simulink model "HVAC_Control_SWC_AUTOSAR_v3_FaultHandling"  (R2022b)
settings: Solver=FixedStepDiscrete  StartTime=0  StopTime=70  FixedStep=0.1  RelTol=1e-3
settings Model: Creator=Utilisateur  LastModifiedBy=Utilisateur
settings DataIOCC: ExternalInput=hvacInputs_SILV3_02  LoadExternalInput=on
settings OptimizationCC: DefaultParameterBehavior=Inlined  UseDivisionForNetSlopeComputation=on  GainParamInheritBuiltInType=on  UseFloatMulNetSlope=on  InlineInvariantSignals=on  EnhancedBackFolding=on  PassReuseOutputArgsAs=Individual arguments  ZeroExternalMemoryAtStartup=off  ZeroInternalMemoryAtStartup=off  NoFixptDivByZeroProtection=on  EfficientFloat2IntCast=on  OptimizeBlockOrder=speed  DifferentSizesBufferReuse=on  OptimizationCustomize=off  EfficientTunableParamExpr=on
settings DebuggingCC: ParameterTunabilityLossMsg=error
settings HardwareCC: ProdLongLongMode=on
settings SFSimCC: MATLABDynamicMemAlloc=off
settings RTWCC: Description=AUTOSAR  SystemTargetFile=autosar.tlc  GenCodeOnly=on  TemplateMakefile=ert_default_tmf
settings CodeAppCC: ForceParamTrailComments=on  IgnoreCustomStorageClasses=off  OperatorAnnotations=on  SimulinkDataObjDesc=on  SFDataObjDesc=on  CustomSymbolStrGlobalVar=rt$N$M  CustomSymbolStrType=$N$M  CustomSymbolStrFcn=$N$M$F  CustomSymbolStrMacro=$N$M  InsertBlockDesc=on
settings STFCustomTargetCC: TargetLangStandard=C99 (ISO)  MultiwordLength=256  ParMdlRefBuildCompliant=on  CompOptLevelCompliant=on  IncludeMdlTerminateFcn=off  CombineOutputUpdateFcns=on  SuppressErrorStatus=on  ERTCustomFileBanners=on  SupportComplex=off  SupportContinuousTime=off  SupportNonInlinedSFcns=off  RemoveResetFunc=on  MATLABClassNameForMDSCustomization=Simulink.SoftwareTarget.ERTCustomization  AutosarCompliant=on  UseToolchainInfoCompliant=on  LookupTableObjectStructAxisOrder=2,1,3,4,...  LUTObjectStructOrderEvenSpacing=Size,Table,Breakpoints  SystemTargetFile=autosar.tlc
settings ERTTargetCC: TargetLangStandard=C99 (ISO)  ConcurrentExecutionCompliant=off  IncludeMdlTerminateFcn=off  SuppressErrorStatus=on  SupportComplex=off  ModelStepFunctionPrototypeControlCompliant=off  CPPClassGenCompliant=off  AutosarCompliant=on  LookupTableObjectStructAxisOrder=2,1,3,4,...  LUTObjectStructOrderEvenSpacing=Size,Table,Breakpoints  InlinedParameterPlacement=NonHierarchical  ERTCustomFileTemplate=example_file_process.tlc

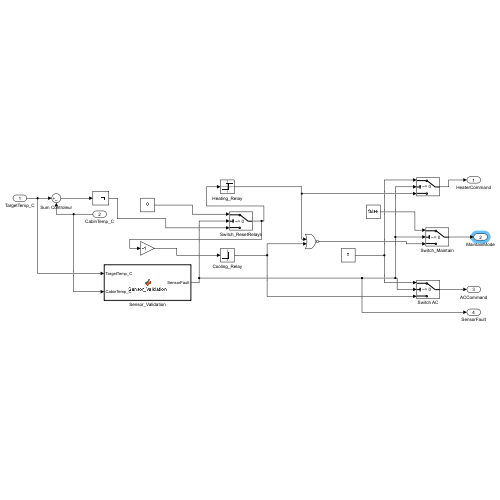
[thumbnail: Simulink's stored preview of the top-level diagram]
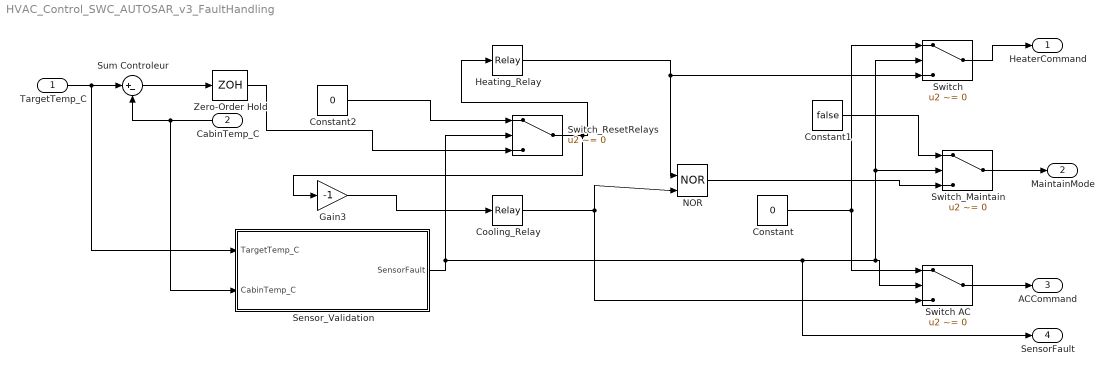
== system HVAC_Control_SWC_AUTOSAR_v3_FaultHandling ==
  TargetTemp_C : Inport
  CabinTemp_C : Inport  Port=2
  Constant : Constant  Value=0
  Constant1 : Constant  Value=false
  Constant2 : Constant  Value=0
  Cooling_Relay : Relay  OnSwitchValue=1  OffSwitchValue=0
  Gain3 : Gain  Gain=-1
  Heating_Relay : Relay  OnSwitchValue=1  OffSwitchValue=0
  NOR : Logic  Operator=NOR  IconShape=distinctive  AllPortsSameDT=off  OutDataTypeStr=boolean
  Sensor_Validation : MATLAB Function  TreatAsAtomicUnit=on
  Sum Controleur : Sum  Inputs=|+-
  Switch : Switch  Criteria=u2 ~= 0  SaturateOnIntegerOverflow=off  InputSameDT=off
  Switch AC : Switch  Criteria=u2 ~= 0  SaturateOnIntegerOverflow=off  InputSameDT=off
  Switch_Maintain : Switch  Criteria=u2 ~= 0  SaturateOnIntegerOverflow=off  InputSameDT=off
  Switch_ResetRelays : Switch  Criteria=u2 ~= 0  SaturateOnIntegerOverflow=off  InputSameDT=off
  Zero-Order Hold : ZeroOrderHold  SampleTime=-1
  HeaterCommand : Outport
  MaintainMode : Outport  Port=2
  ACCommand : Outport  Port=3
  SensorFault : Outport  Port=4
  wires:
  Cooling_Relay/1 -> NOR/2, Switch AC/3
  Sum Controleur/1 -> Zero-Order Hold/1
  Heating_Relay/1 -> NOR/1, Switch/3
  TargetTemp_C/1 -> Sensor_Validation/1(TargetTemp_C), Sum Controleur/1
  Zero-Order Hold/1 -> Switch_ResetRelays/3
  CabinTemp_C/1 -> Sensor_Validation/2(CabinTemp_C), Sum Controleur/2
  Sensor_Validation/1(SensorFault) -> Switch_ResetRelays/2, Switch AC/2, Switch/2, Switch_Maintain/2, SensorFault/1
  Constant/1 -> Switch/1, Switch AC/1
  Switch/1 -> HeaterCommand/1
  Switch AC/1 -> ACCommand/1
  Switch_Maintain/1 -> MaintainMode/1
  NOR/1 -> Switch_Maintain/3
  Constant1/1 -> Switch_Maintain/1
  Constant2/1 -> Switch_ResetRelays/1
  Switch_ResetRelays/1 -> Gain3/1, Heating_Relay/1
  Gain3/1 -> Cooling_Relay/1

== matlab function HVAC_Control_SWC_AUTOSAR_v3_FaultHandling/Sensor_Validation ==
  data: TargetTemp_C input; SensorFault output; CabinTemp_C input

function SensorFault = Sensor_Validation(TargetTemp_C, CabinTemp_C)
%#codegen
% Validation des temperatures HVAC
% SensorFault : double, 0 = valide, 1 = defaut

validTarget = isfinite(TargetTemp_C) && ...
              (TargetTemp_C >= 16) && ...
              (TargetTemp_C <= 30);

validCabin = isfinite(CabinTemp_C) && ...
             (CabinTemp_C >= -20) && ...
             (CabinTemp_C <= 60);

% Conversion explicite boolean vers double
SensorFault = double(~(validTarget && validCabin));

end
